simulink model "s_c_nbe_m32k"  (R2018a)
settings: Solver=VariableStepDiscrete  StartTime=0.0  StopTime=1000  RelTol=1e-3
undefined symbols (not defined in the file): fft_stages, n_taps, output_bits, pfb_coeff_gen_calc, xengbits
libraries: xbsIndex_r4 x23714, casper_library_misc x17, xps_library x4, casper_library_scopes x4, xbsReplacements_r4 x4
(part 10 of 171)

== system s_c_nbe_m32k/cwg_cos ==
  note: If frequency = zero, disable counters
  note: Div 8 as each tick represents 8 samples
  note: 1 = state changed
      | 0 = unchanged
  note: Drop lower 13 bits
  freq : Inport
  scale : Inport  Port=2
  rst : Inport  Port=3
  repeat_en : Inport  Port=4
  repeat_length : Inport  Port=5
  en : Inport  Port=6
  time_in : Inport  Port=7
  AddSub : xbsIndex_r4/AddSub  mode=Subtraction  use_carryin=off  use_carryout=off  en=off  latency=2  precision=Full  arith_type=Unsigned  n_bits=16  bin_pt=14  quantization=Truncate  overflow=Wrap  use_behavioral_HDL=off  hw_selection=Fabric  pipelined=off  dbl_ovrd=off  block_type=addsub
  Constant : xbsIndex_r4/Constant  const=2  gui_display_data_type=Fixed-point  arith_type=Unsigned  n_bits=8  bin_pt=0  preci_type=Single  exp_width=8  frac_width=24  explicit_period=on  period=1  equ=P=C  opselect=C  inp2=PCIN>>17  opr=+  inp1=P  carry=CIN  dbl_ovrd=off  block_type=constant
  Constant1 : xbsIndex_r4/Constant  const=0  gui_display_data_type=Fixed-point  arith_type=Unsigned  n_bits=32  bin_pt=0  preci_type=Single  exp_width=8  frac_width=24  explicit_period=off  period=1  equ=P=C  opselect=C  inp2=PCIN>>17  opr=+  inp1=P  carry=CIN  dbl_ovrd=off  block_type=constant
  Constant2 : xbsIndex_r4/Constant  const=0  gui_display_data_type=Fixed-point  arith_type=Unsigned  n_bits=32  bin_pt=0  preci_type=Single  exp_width=8  frac_width=24  explicit_period=off  period=1  equ=P=C  opselect=C  inp2=PCIN>>17  opr=+  inp1=P  carry=CIN  dbl_ovrd=off  block_type=constant
  Constant3 : xbsIndex_r4/Constant  const=2  gui_display_data_type=Fixed-point  arith_type=Unsigned  n_bits=4  bin_pt=0  preci_type=Single  exp_width=8  frac_width=24  explicit_period=on  period=1  equ=P=C  opselect=C  inp2=PCIN>>17  opr=+  inp1=P  carry=CIN  dbl_ovrd=off  block_type=constant
  Constant4 : xbsIndex_r4/Constant  const=3  gui_display_data_type=Fixed-point  arith_type=Unsigned  n_bits=4  bin_pt=0  preci_type=Single  exp_width=8  frac_width=24  explicit_period=on  period=1  equ=P=C  opselect=C  inp2=PCIN>>17  opr=+  inp1=P  carry=CIN  dbl_ovrd=off  block_type=constant
  Constant5 : xbsIndex_r4/Constant  const=4  gui_display_data_type=Fixed-point  arith_type=Unsigned  n_bits=4  bin_pt=0  preci_type=Single  exp_width=8  frac_width=24  explicit_period=on  period=1  equ=P=C  opselect=C  inp2=PCIN>>17  opr=+  inp1=P  carry=CIN  dbl_ovrd=off  block_type=constant
  Constant6 : xbsIndex_r4/Constant  const=5  gui_display_data_type=Fixed-point  arith_type=Unsigned  n_bits=4  bin_pt=0  preci_type=Single  exp_width=8  frac_width=24  explicit_period=on  period=1  equ=P=C  opselect=C  inp2=PCIN>>17  opr=+  inp1=P  carry=CIN  dbl_ovrd=off  block_type=constant
  Constant7 : xbsIndex_r4/Constant  const=6  gui_display_data_type=Fixed-point  arith_type=Unsigned  n_bits=4  bin_pt=0  preci_type=Single  exp_width=8  frac_width=24  explicit_period=on  period=1  equ=P=C  opselect=C  inp2=PCIN>>17  opr=+  inp1=P  carry=CIN  dbl_ovrd=off  block_type=constant
  Constant8 : xbsIndex_r4/Constant  const=7  gui_display_data_type=Fixed-point  arith_type=Unsigned  n_bits=4  bin_pt=0  preci_type=Single  exp_width=8  frac_width=24  explicit_period=on  period=1  equ=P=C  opselect=C  inp2=PCIN>>17  opr=+  inp1=P  carry=CIN  dbl_ovrd=off  block_type=constant
  Counter : xbsIndex_r4/Counter  cnt_type=Free Running  cnt_to=Inf  operation=Up  start_count=0  cnt_by_val=1  arith_type=Unsigned  n_bits=32  bin_pt=0  load_pin=off  rst=on  en=on  explicit_period=on  period=1  use_behavioral_HDL=off  implementation=Fabric  dbl_ovrd=off  block_type=counter
  Delay : xbsIndex_r4/Delay  rst=off  infoeditControl=Selection of Reset will increase slice count due to use of real FFs and instead of SRLs  en=off  latency=add_latency  reg_retiming=off  dbl_ovrd=off  block_type=delay
  Logical : xbsIndex_r4/Logical  logical_function=OR  inputs=3  en=off  latency=0  precision=Full  arith_type=Unsigned  n_bits=16  bin_pt=0  align_bp=on  dbl_ovrd=off  block_type=logical
  Logical1 : xbsIndex_r4/Logical  logical_function=OR  inputs=2  en=off  latency=0  precision=Full  arith_type=Unsigned  n_bits=16  bin_pt=0  align_bp=on  dbl_ovrd=off  block_type=logical
  Logical2 : xbsIndex_r4/Logical  logical_function=OR  inputs=2  en=off  latency=0  precision=Full  arith_type=Unsigned  n_bits=16  bin_pt=0  align_bp=on  dbl_ovrd=off  block_type=logical
  Logical3 : xbsIndex_r4/Logical  logical_function=AND  inputs=2  en=off  latency=0  precision=Full  arith_type=Unsigned  n_bits=16  bin_pt=0  align_bp=on  dbl_ovrd=off  block_type=logical
  Logical4 : xbsIndex_r4/Logical  logical_function=AND  inputs=2  en=off  latency=0  precision=Full  arith_type=Unsigned  n_bits=16  bin_pt=0  align_bp=on  dbl_ovrd=off  block_type=logical
  Logical5 : xbsIndex_r4/Logical  logical_function=AND  inputs=2  en=off  latency=0  precision=Full  arith_type=Unsigned  n_bits=16  bin_pt=0  align_bp=on  dbl_ovrd=off  block_type=logical
  Mult{,1..13} (14 alike) : xbsIndex_r4/Mult  precision=User Defined  arith_type=Unsigned  n_bits=25+16  bin_pt=0  quantization=Truncate  overflow=Wrap  en=off  latency=mult_latency  use_behavioral_HDL=off  opt=Speed  use_embedded=on  optimum_pipeline=off  pipeline=on  dbl_ovrd=off  use_rpm=on  placement_style=Triangular  block_type=mult
  Register : xbsIndex_r4/Register  init=0  rst=on  en=on  dbl_ovrd=off  block_type=register
  Relational : xbsIndex_r4/Relational  mode=a=b  op_type=Bool  en=off  latency=1  dbl_ovrd=off  block_type=relational
  Relational1 : xbsIndex_r4/Relational  mode=a!=b  op_type=Bool  en=off  latency=1  dbl_ovrd=off  block_type=relational
  Relational2 : xbsIndex_r4/Relational  mode=a!=b  op_type=Bool  en=off  latency=1  dbl_ovrd=off  block_type=relational
  Shift1 : xbsIndex_r4/Shift  shift_dir=Right  shift_bits=3  en=off  latency=0  precision=Full  arith_type="Signed  (2's comp)"  n_bits=16  bin_pt=14  quantization=Truncate  overflow=Wrap  dbl_ovrd=off  block_type=shift
  Slice : xbsIndex_r4/Slice  nbits=28  boolean_output=off  mode=Lower Bit Location + Width  bit1=0  base1=MSB of Input  bit0=0  base0=LSB of Input  dbl_ovrd=off  block_type=slice
  Slice{1..7,9} (8 alike) : xbsIndex_r4/Slice  nbits=13  boolean_output=off  mode=Lower Bit Location + Width  bit1=0  base1=MSB of Input  bit0=9  base0=LSB of Input  dbl_ovrd=off  block_type=slice
  bus_convert : Subsystem  Tag=cmac_delinked  mask(bus_convert){n_bits_in=[34 34 34 34 34 34 34 34], bin_pt_in=32, cmplx=off, n_bits_out=18, bin_pt_out=17, quantization=1, overflow=1, csp_latency=4, of=off, misc=off}
      mask prompts: n_bits_in "input bit widths"; bin_pt_in "input binary points"; cmplx "input complex"; n_bits_out "output bit widths"; bin_pt_out "output binary points"; quantization "quantization strategy (Truncate=0, Round  (unbiased: +/- Inf)=1, Round (unbiased: Even Values)=2)"; overflow "overflow strategy (Wrap=0, Saturate=1, Flag as error=2)"; csp_latency "latency"; of "overflow indication"; misc "misc support"
      mask help: Convert components of busses
      mask init:
      | bus_convert_init(gcb, ...
      |     'n_bits_in', n_bits_in, ...
      |     'bin_pt_in', bin_pt_in, ...
      |     'cmplx', cmplx, ...
      |     'n_bits_out', n_bits_out, ...
      |     'bin_pt_out', bin_pt_out, ...
      |     'quantization', quantization, ...
      |     'overflow', overflow, ...
      |     'csp_latency', csp_latency, ...
      |     'misc', misc, ...
      |     'of', of);
  bus_create : Subsystem  mask(bus_create){inputNum=8}
      mask prompts: inputNum "Number of inputs:"
      mask init:
      | bus_create_init(gcb,...
      |     'inputNum', inputNum);
  bus_mult1 : Subsystem  mask(bus_mult){n_bits_a=[18,18,18,18,18,18,18,18], bin_pt_a=17, type_a=1, cmplx_a=off, n_bits_b=16, bin_pt_b=15, type_b=0, cmplx_b=off, misc=off, floating_point=off, float_type=single, input_vec_a=1, input_vec_b=1, frac_width=19, exp_width=6, n_bits_out=18+16, bin_pt_out=17+15, type_out=1, quantization=1, overflow=1, mult_latency=7, add_latency=7, conv_latency=4, max_fanout=2, fan_latency=3, multiplier_implementation=embedded multiplier core, pipeline_cmult_en=off, pipeline_latency=0}
      mask prompts: n_bits_a "a input bit widths"; bin_pt_a "a input binary points"; type_a "a input type (Unsigned=0, Signed=1)"; cmplx_a "a input complex"; n_bits_b "b input bit widths"; bin_pt_b "b input binary points"; type_b "b input type (Unsigned=0, Signed=1)"; cmplx_b "b input complex"; misc "misc support"; floating_point "floating point"; float_type "float type"; input_vec_a "a input vector in bus"; input_vec_b "b input vector in bus"; frac_width "fraction width"; exp_width "exponent width"; n_bits_out "output bit widths"; bin_pt_out "output binary points"; type_out "output type (Unsigned=0, Signed=1)"; quantization "quantization strategy (Truncate=0, Round  (unbiased: +/- Inf)=1)"; overflow "overflow strategy (Wrap=0, Saturate=1, Flag as error=2)"; mult_latency "multiplier latency"; add_latency "adder latency"; conv_latency "convert latency"; max_fanout "limit fanout to ?"; fan_latency "fanout register latency"; multiplier_implementation "multiplier implementation"; pipeline_cmult_en "pipeline complex mult"; pipeline_latency "pipeline latency"
      mask help: Multiply components of two busses
      mask init: same as s_c_nbe_m32k/DDC/bus_mult
      mask Callback floating_point:
      | onoff = get_param(gcb, 'floating_point');
      | if strcmp(onoff,'on')
      |     enable_fixpt = 'off'
      |     set_param_state(gcb, 'float_type', 'on')
      | 
      |     set_param_state(gcb, 'input_vec_a', 'on')
      |     set_param_state(gcb, 'input_vec_b', 'on')
      | 
      |     f_type = get_param(gcb, 'float_type')
      |     if strcmp(f_type,'custom')
      |         set_param_state(gcb, 'exp_width', 'on')
      |         set_param_state(gcb, 'frac_width', 'on')
      |     else
      |         set_param_state(gcb, 'exp_width', 'off')
      |         set_param_state(gcb, 'frac_width', 'off')
      |     end
      | 
      | else
      |     enable_fixpt = 'on'
      |     set_param_state(gcb, 'float_type', 'off')
      |     set_param_state(gcb, 'exp_width', 'off')
      |     set_param_state(gcb, 'frac_width', 'off')
      |     set_param_state(gcb, 'input_vec_a', 'off')
      |     set_param_state(gcb, 'input_vec_b', 'off')
      | end
      | 
      | set_param_state(gcb, 'n_bits_a', enable_fixpt)
      | set_param_state(gcb, 'bin_pt_a', enable_fixpt)
      | set_param_state(gcb, 'type_a', enable_fixpt)
      | set_param_state(gcb, 'n_bits_b', enable_fixpt)
      | set_param_state(gcb, 'bin_pt_b', enable_fixpt)
      | set_param_state(gcb, 'type_b', enable_fixpt)
      | 
      | set_param_state(gcb, 'n_bits_out', enable_fixpt)
      | set_param_state(gcb, 'bin_pt_out', enable_fixpt)
      | set_param_state(gcb, 'type_out', enable_fixpt)
      | set_param_state(gcb, 'quantization', enable_fixpt)
      | set_param_state(gcb, 'overflow', enable_fixpt)
      mask TypeOptions float_type: single | custom
      mask Callback float_type:
      | f_type = get_param(gcb, 'float_type')
      | if strcmp(f_type,'custom')
      |     set_param_state(gcb, 'exp_width', 'on')
      |     set_param_state(gcb, 'frac_width', 'on')
      | else
      |     set_param_state(gcb, 'exp_width', 'off')
      |     set_param_state(gcb, 'frac_width', 'off')
      | end
      mask TypeOptions multiplier_implementation: behavioral HDL | standard core | embedded multiplier core
      mask Callback pipeline_cmult_en:
      | pipeline_en = get_param(gcb, 'pipeline_cmult_en');
      | if strcmp(pipeline_en,'on')
      | 
      |     set_param_state(gcb, 'pipeline_latency', 'on')
      | else
      |     set_param_state(gcb, 'pipeline_latency', 'off')
      | end
  cosin : Subsystem  Tag=casper:cosin  mask(cosin){output0=cos, output1=cos, indep_theta=on, phase=0, fraction=0, table_bits=13, n_bits=18, bin_pt=17, floating_point=off, float_type=single, exp_width=8, frac_width=24, store=2, pack=off, bram=BRAM, misc=off, bram_latency=10, add_latency=7, mux_latency=2, neg_latency=2, conv_latency=2}
      mask prompts: output0 "first output function"; output1 "second output function"; indep_theta "Independent theta values"; phase "initial phase offset (?*(2*pi))"; fraction "fraction of cycle period to output (1/2^?)"; table_bits "samples in cycle period fraction to output (2^?)"; n_bits "bit width"; bin_pt "binary point"; floating_point "floating point"; float_type "float type"; exp_width "exponent width"; frac_width "fraction width"; store "fraction of cycle period to store (1/2^?)"; pack "pack lookup values in same output word"; bram "BRAM implementation"; misc "Miscellaneous port"; bram_latency "bram latency"; add_latency "large adder latency"; mux_latency "mux latency"; neg_latency "negate latency"; conv_latency "convert latency"
      mask init:
      | cosin_init(gcb, ...
      |     'output0', output0, ...    
      |     'output1', output1, ...
      |     'indep_theta', indep_theta, ...
      |     'phase', phase, ...
      |     'fraction', fraction, ...
      |     'table_bits', table_bits, ...  
      |     'n_bits', n_bits, ...      
      |     'bin_pt', bin_pt, ...    
      |     'floating_point', floating_point, ...
      |     'float_type', float_type, ...
      |     'exp_width', exp_width, ...
      |     'frac_width', frac_width, ...         
      |     'bram_latency', bram_latency, ...
      |     'add_latency', add_latency, ...
      |     'mux_latency', mux_latency, ...
      |     'neg_latency', neg_latency, ...
      |     'conv_latency', conv_latency, ...
      |     'store', store, ...
      |     'pack', pack, ...
      |     'bram', bram, ...
      |     'misc', misc);
      mask TypeOptions output0: sin | cos | -sin | -cos
      mask TypeOptions output1: none | sin | cos | -sin | -cos
      mask Callback floating_point:
      | onoff = get_param(gcb, 'floating_point');
      | if strcmp(onoff,'on')
      |     enable_fixpt = 'off'
      |     set_param_state(gcb, 'float_type', 'on')
      | 
      |     f_type = get_param(gcb, 'float_type')
      |     if strcmp(f_type,'custom')
      |         set_param_state(gcb, 'exp_width', 'on')
      |         set_param_state(gcb, 'frac_width', 'on')
      |     else
      |         set_param_state(gcb, 'exp_width', 'off')
      |         set_param_state(gcb, 'frac_width', 'off')
      |     end
      | 
      | 
      | else
      |     enable_fixpt = 'on'
      |     set_param_state(gcb, 'float_type', 'off')
      |     set_param_state(gcb, 'exp_width', 'off')
      |     set_param_state(gcb, 'frac_width', 'off')
      | end
      | 
      | set_param_state(gcb, 'n_bits', enable_fixpt)
      | set_param_state(gcb, 'bin_pt', enable_fixpt)
      mask TypeOptions float_type: single | custom
      mask Callback float_type:
      | f_type = get_param(gcb, 'float_type')
      | if strcmp(f_type,'custom')
      |     set_param_state(gcb, 'exp_width', 'on')
      |     set_param_state(gcb, 'frac_width', 'on')
      | else
      |     set_param_state(gcb, 'exp_width', 'off')
      |     set_param_state(gcb, 'frac_width', 'off')
      | end
      mask TypeOptions bram: distributed RAM | BRAM
      mask Display:
      | if ~(table_bits == 0),
      |         color('black');port_label('output',1,output0);
      |     color('black');port_label('output',2,output1);
      |     color('black');disp(['z^{-',num2str(add_latency+mux_latency+conv_latency+bram_latency+neg_latency+mux_latency),'}'],'texmode','on');color('black');port_label('input',1,'theta');
      |     if strcmp(misc, 'on'),
      |         color('black');port_label('input',2,'misci');
      |         color('black');port_label('output',3,'misco');
      |     end
      | end
  cosin1 : Subsystem  Tag=casper:cosin  mask(cosin){output0=cos, output1=cos, indep_theta=on, phase=0, fraction=0, table_bits=13, n_bits=18, bin_pt=17, floating_point=off, float_type=single, exp_width=8, frac_width=24, store=2, pack=off, bram=BRAM, misc=off, bram_latency=10, add_latency=7, mux_latency=2, neg_latency=2, conv_latency=2}
      mask prompts: output0 "first output function"; output1 "second output function"; indep_theta "Independent theta values"; phase "initial phase offset (?*(2*pi))"; fraction "fraction of cycle period to output (1/2^?)"; table_bits "samples in cycle period fraction to output (2^?)"; n_bits "bit width"; bin_pt "binary point"; floating_point "floating point"; float_type "float type"; exp_width "exponent width"; frac_width "fraction width"; store "fraction of cycle period to store (1/2^?)"; pack "pack lookup values in same output word"; bram "BRAM implementation"; misc "Miscellaneous port"; bram_latency "bram latency"; add_latency "large adder latency"; mux_latency "mux latency"; neg_latency "negate latency"; conv_latency "convert latency"
      mask init: same as s_c_nbe_m32k/cwg_cos/cosin
      mask TypeOptions output0: sin | cos | -sin | -cos
      mask TypeOptions output1: none | sin | cos | -sin | -cos
      mask Callback floating_point:
      | onoff = get_param(gcb, 'floating_point');
      | if strcmp(onoff,'on')
      |     enable_fixpt = 'off'
      |     set_param_state(gcb, 'float_type', 'on')
      | 
      |     f_type = get_param(gcb, 'float_type')
      |     if strcmp(f_type,'custom')
      |         set_param_state(gcb, 'exp_width', 'on')
      |         set_param_state(gcb, 'frac_width', 'on')
      |     else
      |         set_param_state(gcb, 'exp_width', 'off')
      |         set_param_state(gcb, 'frac_width', 'off')
      |     end
      | 
      | 
      | else
      |     enable_fixpt = 'on'
      |     set_param_state(gcb, 'float_type', 'off')
      |     set_param_state(gcb, 'exp_width', 'off')
      |     set_param_state(gcb, 'frac_width', 'off')
      | end
      | 
      | set_param_state(gcb, 'n_bits', enable_fixpt)
      | set_param_state(gcb, 'bin_pt', enable_fixpt)
      mask TypeOptions float_type: single | custom
      mask Callback float_type:
      | f_type = get_param(gcb, 'float_type')
      | if strcmp(f_type,'custom')
      |     set_param_state(gcb, 'exp_width', 'on')
      |     set_param_state(gcb, 'frac_width', 'on')
      | else
      |     set_param_state(gcb, 'exp_width', 'off')
      |     set_param_state(gcb, 'frac_width', 'off')
      | end
      mask TypeOptions bram: distributed RAM | BRAM
      mask Display:
      | if ~(table_bits == 0),
      |         color('black');port_label('output',1,output0);
      |     color('black');port_label('output',2,output1);
      |     color('black');disp(['z^{-',num2str(add_latency+mux_latency+conv_latency+bram_latency+neg_latency+mux_latency),'}'],'texmode','on');color('black');port_label('input',1,'theta');
      |     if strcmp(misc, 'on'),
      |         color('black');port_label('input',2,'misci');
      |         color('black');port_label('output',3,'misco');
      |     end
      | end
  cosin2 : Subsystem  Tag=casper:cosin  mask(cosin){output0=cos, output1=cos, indep_theta=on, phase=0, fraction=0, table_bits=13, n_bits=18, bin_pt=17, floating_point=off, float_type=single, exp_width=8, frac_width=24, store=2, pack=off, bram=BRAM, misc=off, bram_latency=10, add_latency=7, mux_latency=2, neg_latency=2, conv_latency=2}
      mask prompts: output0 "first output function"; output1 "second output function"; indep_theta "Independent theta values"; phase "initial phase offset (?*(2*pi))"; fraction "fraction of cycle period to output (1/2^?)"; table_bits "samples in cycle period fraction to output (2^?)"; n_bits "bit width"; bin_pt "binary point"; floating_point "floating point"; float_type "float type"; exp_width "exponent width"; frac_width "fraction width"; store "fraction of cycle period to store (1/2^?)"; pack "pack lookup values in same output word"; bram "BRAM implementation"; misc "Miscellaneous port"; bram_latency "bram latency"; add_latency "large adder latency"; mux_latency "mux latency"; neg_latency "negate latency"; conv_latency "convert latency"
      mask init: same as s_c_nbe_m32k/cwg_cos/cosin
      mask TypeOptions output0: sin | cos | -sin | -cos
      mask TypeOptions output1: none | sin | cos | -sin | -cos
      mask Callback floating_point:
      | onoff = get_param(gcb, 'floating_point');
      | if strcmp(onoff,'on')
      |     enable_fixpt = 'off'
      |     set_param_state(gcb, 'float_type', 'on')
      | 
      |     f_type = get_param(gcb, 'float_type')
      |     if strcmp(f_type,'custom')
      |         set_param_state(gcb, 'exp_width', 'on')
      |         set_param_state(gcb, 'frac_width', 'on')
      |     else
      |         set_param_state(gcb, 'exp_width', 'off')
      |         set_param_state(gcb, 'frac_width', 'off')
      |     end
      | 
      | 
      | else
      |     enable_fixpt = 'on'
      |     set_param_state(gcb, 'float_type', 'off')
      |     set_param_state(gcb, 'exp_width', 'off')
      |     set_param_state(gcb, 'frac_width', 'off')
      | end
      | 
      | set_param_state(gcb, 'n_bits', enable_fixpt)
      | set_param_state(gcb, 'bin_pt', enable_fixpt)
      mask TypeOptions float_type: single | custom
      mask Callback float_type:
      | f_type = get_param(gcb, 'float_type')
      | if strcmp(f_type,'custom')
      |     set_param_state(gcb, 'exp_width', 'on')
      |     set_param_state(gcb, 'frac_width', 'on')
      | else
      |     set_param_state(gcb, 'exp_width', 'off')
      |     set_param_state(gcb, 'frac_width', 'off')
      | end
      mask TypeOptions bram: distributed RAM | BRAM
      mask Display:
      | if ~(table_bits == 0),
      |         color('black');port_label('output',1,output0);
      |     color('black');port_label('output',2,output1);
      |     color('black');disp(['z^{-',num2str(add_latency+mux_latency+conv_latency+bram_latency+neg_latency+mux_latency),'}'],'texmode','on');color('black');port_label('input',1,'theta');
      |     if strcmp(misc, 'on'),
      |         color('black');port_label('input',2,'misci');
      |         color('black');port_label('output',3,'misco');
      |     end
      | end
  cosin3 : Subsystem  Tag=casper:cosin  mask(cosin){output0=cos, output1=cos, indep_theta=on, phase=0, fraction=0, table_bits=13, n_bits=18, bin_pt=17, floating_point=off, float_type=single, exp_width=8, frac_width=24, store=2, pack=off, bram=BRAM, misc=off, bram_latency=10, add_latency=7, mux_latency=2, neg_latency=2, conv_latency=2}
      mask prompts: output0 "first output function"; output1 "second output function"; indep_theta "Independent theta values"; phase "initial phase offset (?*(2*pi))"; fraction "fraction of cycle period to output (1/2^?)"; table_bits "samples in cycle period fraction to output (2^?)"; n_bits "bit width"; bin_pt "binary point"; floating_point "floating point"; float_type "float type"; exp_width "exponent width"; frac_width "fraction width"; store "fraction of cycle period to store (1/2^?)"; pack "pack lookup values in same output word"; bram "BRAM implementation"; misc "Miscellaneous port"; bram_latency "bram latency"; add_latency "large adder latency"; mux_latency "mux latency"; neg_latency "negate latency"; conv_latency "convert latency"
      mask init: same as s_c_nbe_m32k/cwg_cos/cosin
      mask TypeOptions output0: sin | cos | -sin | -cos
      mask TypeOptions output1: none | sin | cos | -sin | -cos
      mask Callback floating_point:
      | onoff = get_param(gcb, 'floating_point');
      | if strcmp(onoff,'on')
      |     enable_fixpt = 'off'
      |     set_param_state(gcb, 'float_type', 'on')
      | 
      |     f_type = get_param(gcb, 'float_type')
      |     if strcmp(f_type,'custom')
      |         set_param_state(gcb, 'exp_width', 'on')
      |         set_param_state(gcb, 'frac_width', 'on')
      |     else
      |         set_param_state(gcb, 'exp_width', 'off')
      |         set_param_state(gcb, 'frac_width', 'off')
      |     end
      | 
      | 
      | else
      |     enable_fixpt = 'on'
      |     set_param_state(gcb, 'float_type', 'off')
      |     set_param_state(gcb, 'exp_width', 'off')
      |     set_param_state(gcb, 'frac_width', 'off')
      | end
      | 
      | set_param_state(gcb, 'n_bits', enable_fixpt)
      | set_param_state(gcb, 'bin_pt', enable_fixpt)
      mask TypeOptions float_type: single | custom
      mask Callback float_type:
      | f_type = get_param(gcb, 'float_type')
      | if strcmp(f_type,'custom')
      |     set_param_state(gcb, 'exp_width', 'on')
      |     set_param_state(gcb, 'frac_width', 'on')
      | else
      |     set_param_state(gcb, 'exp_width', 'off')
      |     set_param_state(gcb, 'frac_width', 'off')
      | end
      mask TypeOptions bram: distributed RAM | BRAM
      mask Display:
      | if ~(table_bits == 0),
      |         color('black');port_label('output',1,output0);
      |     color('black');port_label('output',2,output1);
      |     color('black');disp(['z^{-',num2str(add_latency+mux_latency+conv_latency+bram_latency+neg_latency+mux_latency),'}'],'texmode','on');color('black');port_label('input',1,'theta');
      |     if strcmp(misc, 'on'),
      |         color('black');port_label('input',2,'misci');
      |         color('black');port_label('output',3,'misco');
      |     end
      | end
  edge_detect : Subsystem  mask(edge_detect){edge=Both, polarity=Active High, x_in=[0 0.08 0.08 0.16 0.16 0.24 0.24 0.32 0.32 0.4], y_in=[-1 -1  1  1  1  1  1  1  1  1], x_out=[0.6 0.68 0.68 0.76 0.76 0.84 0.84 0.92 0.92 1], y_out=[-1 -1  1  1 -1 -1 -1 -1 -1 -1]}
      mask prompts: edge "Edge Type"; polarity "Output Polarity"; x_in "Input X Positions"; y_in "Input Y Positions"; x_out "Output X Positions"; y_out "Output Y Positions"
      mask help: Output is active for one-cycle after each edge of the specified type (i.e. rising, falling or both).
      mask init: same as s_c_nbe_m32k/edge_detect1
      settings: AttributesFormatString=|
      | both edges
      | active high
      mask Help: Output is active for one-cycle after each edge of the specified type (i.e. rising, falling, or both).  Latency is zero.
      mask TypeOptions edge: Rising | Falling | Both
      mask TypeOptions polarity: Active High | Active Low
      mask Display:
      | plot(x_in_num,0.5+y_in_num*0.2);
      | plot(x_out_num,0.5+y_out_num*0.2);
  edge_detect1 : Subsystem  mask(edge_detect){edge=Rising, polarity=Active High, x_in=[0 0.08 0.08 0.16 0.16 0.24 0.24 0.32 0.32 0.4], y_in=[-1 -1  1  1  1  1  1  1  1  1], x_out=[0.6 0.68 0.68 0.76 0.76 0.84 0.84 0.92 0.92 1], y_out=[-1 -1  1  1 -1 -1 -1 -1 -1 -1]}
      mask prompts: edge "Edge Type"; polarity "Output Polarity"; x_in "Input X Positions"; y_in "Input Y Positions"; x_out "Output X Positions"; y_out "Output Y Positions"
      mask help: Output is active for one-cycle after each edge of the specified type (i.e. rising, falling or both).
      mask init: same as s_c_nbe_m32k/edge_detect1
      settings: AttributesFormatString=|
      | rising edges
      | active high
      mask Help: Output is active for one-cycle after each edge of the specified type (i.e. rising, falling, or both).  Latency is zero.
      mask TypeOptions edge: Rising | Falling | Both
      mask TypeOptions polarity: Active High | Active Low
      mask Display:
      | plot(x_in_num,0.5+y_in_num*0.2);
      | plot(x_out_num,0.5+y_out_num*0.2);
  offset_sum{1..7} (7 alike) : xbsIndex_r4/AddSub  mode=Addition  use_carryin=off  use_carryout=off  en=off  latency=add_latency  precision=User Defined  arith_type=Unsigned  n_bits=25+16  bin_pt=0  quantization=Truncate  overflow=Wrap  use_behavioral_HDL=off  hw_selection=Fabric  pipelined=on  use_rpm=on  dbl_ovrd=off  block_type=addsub
      settings: block_version=10.1.3
  pipeline10 : Subsystem  Tag=cmac_delinked  mask(pipeline){csp_latency=1}
      mask prompts: csp_latency "Latency"
      mask help:
      | An explicitly laid-out delay line to avoid mapping to SRL16s
      | for use in pipelining to help achieve timing closure.
      mask init:
      | pipeline_init(gcb,'latency',csp_latency);
      settings: AttributesFormatString=Latency = %<latency>
      mask Display:
      | port_label('input', 1, 'd');
      | port_label('output', 1, 'q');
      | disp(['Z^-', num2str(csp_latency)]);
  pipeline41 : Subsystem  Tag=cmac_delinked  mask(pipeline){csp_latency=2}
      mask prompts: csp_latency "Latency"
      mask help:
      | An explicitly laid-out delay line to avoid mapping to SRL16s
      | for use in pipelining to help achieve timing closure.
      mask init:
      | pipeline_init(gcb,'latency',csp_latency);
      settings: AttributesFormatString=Latency = %<latency>
      mask Display:
      | port_label('input', 1, 'd');
      | port_label('output', 1, 'q');
      | disp(['Z^-', num2str(csp_latency)]);
  pipeline8 : Subsystem  Tag=cmac_delinked  mask(pipeline){csp_latency=2}
      mask prompts: csp_latency "Latency"
      mask help:
      | An explicitly laid-out delay line to avoid mapping to SRL16s
      | for use in pipelining to help achieve timing closure.
      mask init:
      | pipeline_init(gcb,'latency',csp_latency);
      settings: AttributesFormatString=Latency = %<latency>
      mask Display:
      | port_label('input', 1, 'd');
      | port_label('output', 1, 'q');
      | disp(['Z^-', num2str(csp_latency)]);
  pipeline9 : Subsystem  Tag=cmac_delinked  mask(pipeline){csp_latency=1}
      mask prompts: csp_latency "Latency"
      mask help:
      | An explicitly laid-out delay line to avoid mapping to SRL16s
      | for use in pipelining to help achieve timing closure.
      mask init:
      | pipeline_init(gcb,'latency',csp_latency);
      settings: AttributesFormatString=Latency = %<latency>
      mask Display:
      | port_label('input', 1, 'd');
      | port_label('output', 1, 'q');
      | disp(['Z^-', num2str(csp_latency)]);
  register_change_detect : Subsystem
  bus_out : Outport
  dvalid : Outport  Port=2
  rpt_rst : Outport  Port=3
  wires:
  Slice3/1 -> cosin2/2(theta2)
  Mult8/1 -> offset_sum5/1
  Constant5/1 -> Mult6/1
  Constant6/1 -> Mult8/1
  Mult9/1 -> offset_sum5/2
  Slice6/1 -> cosin3/1(theta)
  Mult6/1 -> offset_sum4/1
  Mult5/1 -> offset_sum3/2
  Slice5/1 -> cosin1/2(theta2)
  Mult1/1 -> offset_sum1/2
  offset_sum2/1 -> Slice4/1
  Mult3/1 -> offset_sum2/2
  Constant3/1 -> Mult2/1
  [time_in_28] -> Mult1/1
  Mult7/1 -> offset_sum4/2
  [time_in_28] -> Mult11/1
  freq/1 -> Relational2/1, Mult/2, Mult1/2, offset_sum1/1, Mult2/2, Mult3/2, Mult5/2, Mult4/2, Mult7/2, Mult6/2, Mult8/2, Mult9/2, Mult11/2, Mult10/2, Mult13/2, Mult12/2, register_change_detect/1(data)
  Mult10/1 -> offset_sum6/1
  Slice7/1 -> cosin3/2(theta2)
  Mult12/1 -> offset_sum7/1
  Constant7/1 -> Mult10/1
  Constant8/1 -> Mult12/1
  Mult11/1 -> offset_sum6/2
  Mult13/1 -> offset_sum7/2
  Mult/1 -> Delay/1
  [time_in_28] -> Mult/1
  Mult4/1 -> offset_sum3/1
  Mult2/1 -> offset_sum2/1
  Constant4/1 -> Mult4/1
  Slice1/1 -> cosin/2(theta2)
  cosin/2(cos1) -> bus_create/2(in2)
  cosin/1(cos0) -> bus_create/1(in1)
  bus_create/1(bus_out) -> pipeline41/1(d)
  scale/1 -> bus_mult1/2(b)
  pipeline41/1(q) -> bus_mult1/1(a)
  cosin3/1(cos0) -> bus_create/7(in7)
  cosin1/1(cos0) -> bus_create/3(in3)
  cosin1/2(cos1) -> bus_create/4(in4)
  cosin2/1(cos0) -> bus_create/5(in5)
  cosin2/2(cos1) -> bus_create/6(in6)
  bus_mult1/1(a*b) -> bus_convert/1(din)
  Slice2/1 -> cosin2/1(theta)
  Slice9/1 -> cosin/1(theta)
  Delay/1 -> Slice9/1
  offset_sum1/1 -> Slice1/1
  offset_sum3/1 -> Slice5/1
  offset_sum4/1 -> Slice2/1
  offset_sum5/1 -> Slice3/1
  offset_sum6/1 -> Slice6/1
  offset_sum7/1 -> Slice7/1
  Logical/1 -> Register/2
  edge_detect/1(out) -> Logical/1
  Counter/1 -> Relational/1
  rst/1 -> [rst_local]
  Logical1/1 -> Counter/1
  [rst_local] -> Logical1/1
  [rst_cntrs] -> Logical1/2
  [rst_local] -> register_change_detect/2(rst)
  [rst_local] -> Logical/2
  register_change_detect/1(state_change) -> pipeline9/1(d), edge_detect/1(in)
  edge_detect1/1(out) -> Logical/3
  Relational/1 -> pipeline10/1(d), edge_detect1/1(in), rpt_rst/1, [rst_cntrs]
  repeat_length/1 -> Relational1/1, Shift1/1
  AddSub/1 -> Relational/2
  Constant/1 -> AddSub/2
  bus_convert/1(dout) -> pipeline8/1(d)
  pipeline9/1(q) -> Logical2/1
  pipeline10/1(q) -> Logical2/2
  pipeline8/1(q) -> bus_out/1
  [en] -> register_change_detect/3(en)
  Shift1/1 -> AddSub/1
  repeat_en/1 -> Logical3/1
  Logical3/1 -> Counter/2
  Relational1/1 -> Logical3/2
  Constant1/1 -> Relational1/2
  Constant2/1 -> Relational2/2
  Relational2/1 -> Logical4/1
  en/1 -> Logical4/2, [en]
  Logical4/1 -> [en_cntrs]
  [en_cntrs] -> Logical5/2
  Logical2/1 -> Logical5/1
  Logical5/1 -> Register/1, Register/3
  Slice4/1 -> cosin1/1(theta)
  Register/1 -> dvalid/1
  cosin3/2(cos1) -> bus_create/8(in8)
  time_in/1 -> Slice/1
  [time_in_28] -> Mult3/1
  [time_in_28] -> Mult5/1
  [time_in_28] -> Mult7/1
  [time_in_28] -> Mult9/1
  [time_in_28] -> Mult13/1
  Slice/1 -> [time_in_28]
